simulink model "TP3_reprise_commande_des_retroviseurs_StateFlow"  (R2022b)
settings: Solver=VariableStepAuto  StartTime=0.0  StopTime=inf  RelTol=1e-3
settings Model: Creator=HP  LastModifiedBy=HP

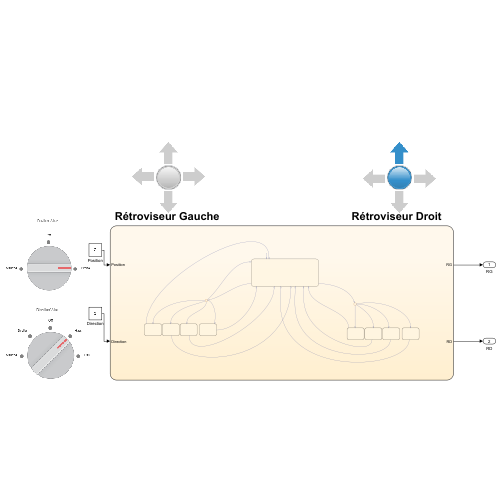
[thumbnail: Simulink's stored preview of the top-level diagram]
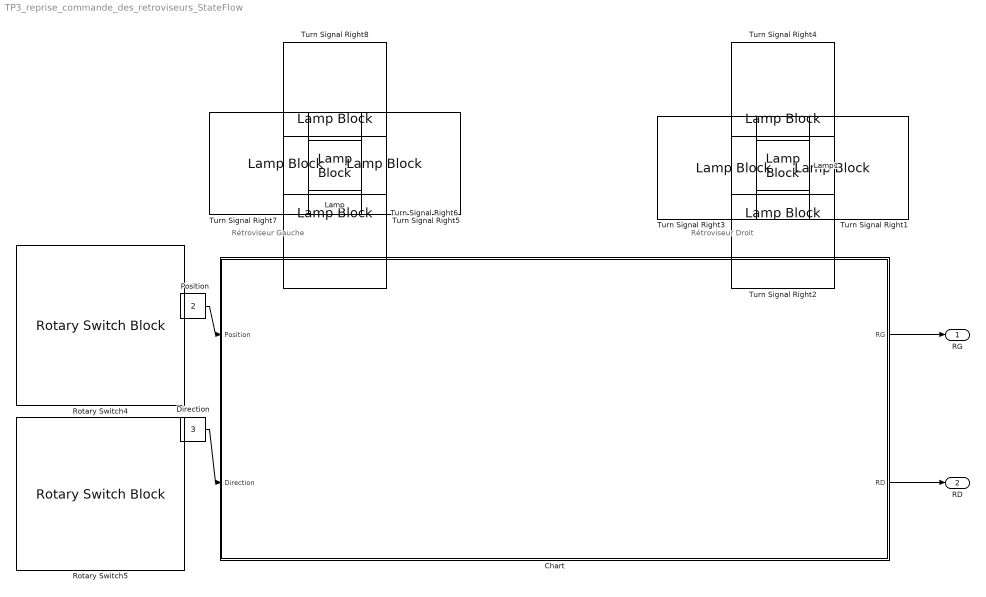
== system TP3_reprise_commande_des_retroviseurs_StateFlow ==
  note: Rétroviseur Droit
  note: Rétroviseur Gauche
  Chart : Stateflow chart  TreatAsAtomicUnit=on
  Direction : Constant  Value=3
  Lamp : LampBlock  LabelPosition=Hide
  Lamp1 : LampBlock  LabelPosition=Hide
  Position : Constant  Value=2
  Rotary Switch4 : RotarySwitchBlock
      settings: Values={{'Gauche', 'Off', 'Droite'}, [1 0 2]}
  Rotary Switch5 : RotarySwitchBlock
      settings: Values={{'Gauche', 'Droite', 'Off', 'Haut', 'Bas'}, [1 2 0 3 4]}
  Turn Signal Right{1..8} (8 alike) : LampBlock  LabelPosition=Hide  Icon=TurnSignalRight
  RG : Outport
  RD : Outport  Port=2
  wires:
  Position/1 -> Chart/1(Position)
  Direction/1 -> Chart/2(Direction)
  Chart/2(RD) -> RD/1
  Chart/1(RG) -> RG/1

== stateflow chart TP3_reprise_commande_des_retroviseurs_StateFlow/Chart ==
  state Repos
    entry:
    RG = 0;
    RD = 0;
  state Gauche_Ouest
    entry:
    RG = 1;
    RD = 0;
  state Gauche_Est
    entry:
    RG = 2;
    RD = 0;
  state Gauche_Nord
    entry:
    RG = 3;
    RD = 0;
  state Gauche_Sud
    entry:
    RG = 4;
    RD = 0;
  state Droite_Ouest
    entry:
    RG = 0;
    RD = 1;
  state Droite_Est
    entry:
    RG = 0;
    RD = 2;
  state Droite_Nord
    entry:
    RG = 0;
    RD = 3;
  state Droite_Sud
    entry:
    RG = 0;
    RD = 4;
  Gauche_Ouest -> Repos : [Direction ~=1 || Position ~= 1]
  (default) -> Repos
  (junction 12) -> Repos [order 1] : [Position ==0]
  Repos -> (junction 12) [order 1] : [Position == 1]
  Repos -> (junction 13) [order 2] : [Position == 2]
  Gauche_Est -> Repos : [Direction ~= 2 || Position ~= 1]
  Gauche_Nord -> Repos : [Direction ~= 3 || Position ~= 1]
  Gauche_Sud -> Repos : [Direction ~= 4 || Position ~= 1]
  Droite_Sud -> Repos : [Direction ~= 4 || Position ~= 2]
  Droite_Nord -> Repos : [Direction ~= 3 || Position ~= 2]
  Droite_Est -> Repos : [Direction ~= 2 || Position ~= 2]
  Droite_Ouest -> Repos : [Direction ~= 1 || Position ~= 2]
  (junction 12) -> Gauche_Ouest [order 5] : [Direction == 1]
  (junction 12) -> Gauche_Sud [order 3] : [Direction == 4]
  (junction 12) -> Gauche_Est [order 2] : [Direction == 2]
  (junction 12) -> Gauche_Nord [order 4] : [Direction == 3]
  (junction 13) -> Droite_Sud [order 3] : [Direction == 4]
  (junction 13) -> Droite_Nord [order 2] : [Direction == 3]
  (junction 13) -> Droite_Est [order 1] : [Direction == 2]
  (junction 13) -> Droite_Ouest [order 4] : [Direction == 1]
  data: RG output; Position input; Direction input; RD output
